simulink model "Engine_Speed_Control"  (R2025a)
settings: Solver=VariableStepAuto  StartTime=0.0  StopTime=10.0  RelTol=1e-3
settings Model: Creator=nikul  LastModifiedBy=nikul

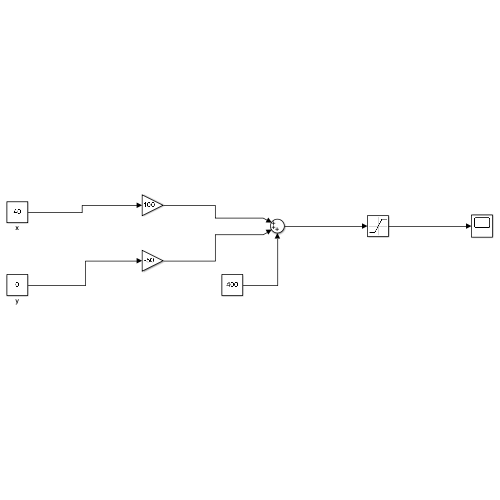
[thumbnail: Simulink's stored preview of the top-level diagram]
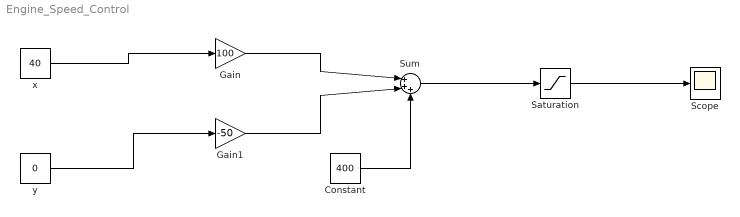
== system Engine_Speed_Control ==
  Constant : Constant  Value=400
  Gain : Gain  Gain=100
  Gain1 : Gain  Gain=-50
  Saturation : Saturate  UpperLimit=3000  LowerLimit=100
  Scope : Scope
      settings: ActiveDisplayYMinimum=2000  ActiveDisplayYMaximum=4000
  Sum : Sum  Inputs=|+++
  x : Constant  Value=40
  y : Constant  Value=0
  wires:
  x/1 -> Gain/1
  y/1 -> Gain1/1
  Gain/1 -> Sum/1
  Gain1/1 -> Sum/2
  Constant/1 -> Sum/3
  Sum/1 -> Saturation/1
  Saturation/1 -> Scope/1
